simulink model "ilqar_lab4"  (R2026b)
settings: Solver=VariableStepAuto
libraries: dspfdesign x7
settings Model: Creator=Campus415  LastModifiedBy=ilqar

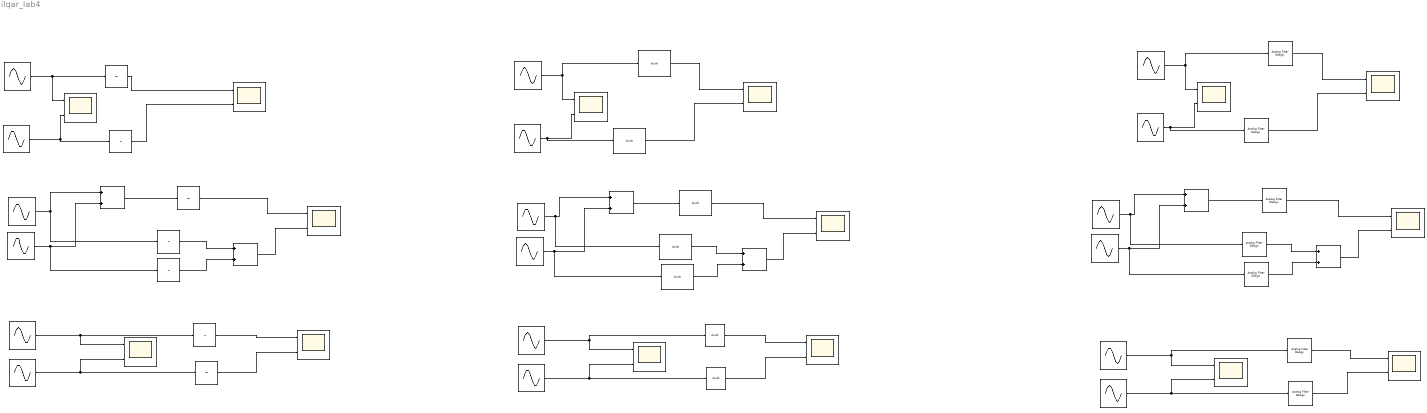
== system ilqar_lab4 ==
  note: INTEGRATOR
  note: Additivity
  note: Homogenity
  note: Shift Invariance
  note: Before Integration
  note: After Integration
  note: DERIVATIVE
  note: Before Derivation
  note: After Derivation
  note: Additivity
  note: Shift Invariance
  note: FILTER
  note: Before FIiltering
  note: After Filtering
  note: Additivity
  note: Shift Invariance
  Add{,1..5} (6 alike) : Sum
  Analog Filter Design{,1..6} (7 alike) : dspfdesign/Analog Filter Design  method=Butterworth  filttype=Lowpass  N=8  Wlo=30  Whi=80  Rp=2  Rs=40
  Derivative{,1..6} (7 alike) : Derivative
  Integrator{,1..6} (7 alike) : Integrator
  Scope{,1..14} (15 alike) : Scope  NumInputPorts=2
      Scope settings: ActiveDisplayYMinimum=-0.53193054239870508  ActiveDisplayYMaximum=4.7172636926188911
      Scope1 settings: ActiveDisplayYMinimum=-1  ActiveDisplayYMaximum=1
      Scope10 settings: ActiveDisplayYMinimum=-1.8295977325680854  ActiveDisplayYMaximum=9.6287349725327882  DataLoggingVariableName=ScopeData10
      Scope11 settings: ActiveDisplayYMinimum=-2.4977432196827314  ActiveDisplayYMaximum=2.4995360011907284  DataLoggingVariableName=ScopeData11
      Scope12 settings: ActiveDisplayYMinimum=-0.7498848907167992  ActiveDisplayYMaximum=6.7489640164511941  DataLoggingVariableName=ScopeData12
      Scope13 settings: ActiveDisplayYMinimum=-1.8011727234255441  ActiveDisplayYMaximum=2.8874722573589677  DataLoggingVariableName=ScopeData13
      Scope14 settings: ActiveDisplayYMinimum=-1.2488716092982026  ActiveDisplayYMaximum=2.2498674647262433  DataLoggingVariableName=ScopeData14
      Scope2 settings: ActiveDisplayYMinimum=-0.7498848907167992  ActiveDisplayYMaximum=6.7489640164511941  DataLoggingVariableName=ScopeData2
      Scope3 settings: ActiveDisplayYMinimum=-1.8011727234255441  ActiveDisplayYMaximum=2.8874722573589677  DataLoggingVariableName=ScopeData3
      Scope4 settings: ActiveDisplayYMinimum=-1.2488716092982026  ActiveDisplayYMaximum=2.2498674647262433  DataLoggingVariableName=ScopeData4
      Scope5 settings: ActiveDisplayYMinimum=-1.8295977325680854  ActiveDisplayYMaximum=9.6287349725327882  DataLoggingVariableName=ScopeData5
      Scope6 settings: ActiveDisplayYMinimum=-1  ActiveDisplayYMaximum=1  DataLoggingVariableName=ScopeData6
      Scope7 settings: ActiveDisplayYMinimum=-0.7498848907167992  ActiveDisplayYMaximum=6.7489640164511941  DataLoggingVariableName=ScopeData7
      Scope8 settings: ActiveDisplayYMinimum=-1.8011727234255441  ActiveDisplayYMaximum=2.8874722573589677  DataLoggingVariableName=ScopeData8
      Scope9 settings: ActiveDisplayYMinimum=-1.2488716092982026  ActiveDisplayYMaximum=2.2498674647262433  DataLoggingVariableName=ScopeData9
  Sine Wave{,2,4,6,8,10,12,14,16} (9 alike) : Sin  SampleTime=0
  Sine Wave{1,3,7,9,13,15} (6 alike) : Sin  Amplitude=2  SampleTime=0
  Sine Wave11 : Sin  Phase=pi/2  SampleTime=0
  Sine Wave17 : Sin  Phase=pi/2  SampleTime=0
  Sine Wave5 : Sin  Phase=pi/2  SampleTime=0
  wires:
  Sine Wave/1 -> Scope1/1, Integrator/1
  Integrator/1 -> Scope/1
  Sine Wave1/1 -> Scope1/2, Integrator1/1
  Integrator1/1 -> Scope/2
  Sine Wave2/1 -> Integrator3/1, Add/1
  Sine Wave3/1 -> Integrator4/1, Add/2
  Add/1 -> Integrator2/1
  Integrator2/1 -> Scope2/1
  Integrator3/1 -> Add1/1
  Integrator4/1 -> Add1/2
  Add1/1 -> Scope2/2
  Sine Wave4/1 -> Scope4/1, Integrator5/1
  Sine Wave5/1 -> Scope4/2, Integrator6/1
  Integrator5/1 -> Scope3/1
  Integrator6/1 -> Scope3/2
  Sine Wave7/1 -> Derivative1/1, Scope6/2
  Derivative/1 -> Scope5/1
  Sine Wave6/1 -> Scope6/1, Derivative/1
  Derivative1/1 -> Scope5/2
  Derivative6/1 -> Scope8/2
  Derivative5/1 -> Scope8/1
  Sine Wave11/1 -> Scope9/2, Derivative6/1
  Sine Wave10/1 -> Derivative5/1, Scope9/1
  Add3/1 -> Scope7/2
  Sine Wave9/1 -> Derivative4/1, Add2/2
  Sine Wave8/1 -> Derivative3/1, Add2/1
  Derivative3/1 -> Add3/1
  Derivative4/1 -> Add3/2
  Add2/1 -> Derivative2/1
  Derivative2/1 -> Scope7/1
  Analog Filter Design1/1 -> Scope10/2
  Sine Wave12/1 -> Analog Filter Design/1, Scope11/1
  Analog Filter Design/1 -> Scope10/1
  Sine Wave13/1 -> Analog Filter Design1/1, Scope11/2
  Analog Filter Design2/1 -> Scope12/1
  Add4/1 -> Analog Filter Design2/1
  Analog Filter Design4/1 -> Add5/2
  Analog Filter Design3/1 -> Add5/1
  Sine Wave14/1 -> Analog Filter Design3/1, Add4/1
  Sine Wave15/1 -> Analog Filter Design4/1, Add4/2
  Add5/1 -> Scope12/2
  Sine Wave16/1 -> Analog Filter Design5/1, Scope14/1
  Sine Wave17/1 -> Analog Filter Design6/1, Scope14/2
  Analog Filter Design6/1 -> Scope13/2
  Analog Filter Design5/1 -> Scope13/1
